simulink model "ieee14_fault"  (R2025b)
settings: Solver=ode23t  StartTime=0.0  StopTime=0.12  FixedStep=0.2  RelTol=1e-4  AbsTol=1e-6  EnableMultiTasking=on
undefined symbols (not defined in the file or in its folder): D1, Delta
libraries: spsDiodeLib x84, spsGroundLib x84, spsSeriesRLCBranchLib x84, spsDCVoltageSourceLib x84, spsBreakerLib x42, spsThreePhaseSeriesRLCBranchLib x20, spsThreePhaseVIMeasurementLib x16, spsThreePhaseFaultLib x14, spsThreePhaseSeriesRLCLoadLib x11, spsThreePhaseSourceLib x5, spsThreePhaseTransformerTwoWindingsLib x5, spspowerguiLib x1
(part 1 of 3)
settings Model: Creator=Bharath  LastModifiedBy=ubuntu
settings SolverCC: AutoScaleAbsTol=off  MaxConsecutiveMinStep=auto  ZeroCrossControl=DisableAll  AlgebraicLoopSolver=TrustRegion
settings DataIOCC: LimitDataPoints=on  SaveFormat=Array  SignalLoggingSaveFormat=ModelDataLogs  ReturnWorkspaceOutputs=off
settings OptimizationCC: ExpressionDepthLimit=2147483647.0  LifeSpan=inf
settings DebuggingCC: UnderspecifiedInitializationDetection=Classic  MergeDetectMultiDrivingBlocksExec=none  FcnCallInpInsideContextMsg=warning  UnconnectedInputMsg=warning  UnconnectedLineMsg=warning  StateNameClashWarn=warning  SFUnexpectedBacktrackingDiag=warning  SFNoUnconditionalDefaultTransitionDiag=warning  SFExecutionAtInitializationDiag=none  ArithmeticOperatorsInVariantConditions=warning
settings HardwareCC: ProdBitPerPointer=32.0  ProdBitPerSizeT=32.0  ProdBitPerPtrDiffT=32.0  ProdLargestAtomicFloat=None  ProdIntDivRoundTo=Undefined  ProdEndianess=Unspecified  ProdWordSize=32.0  ProdHWDeviceType=32-bit Generic
settings ModelReferenceCC: PropagateSignalLabelsOutOfModel=off
settings SFSimCC: SimUseLocalCustomCode=off  CustomCodeUndefinedFunction=UseInterfaceOnly
settings RTWCC: RTWUseLocalCustomCode=off  GPUComputeCapability=3.5
settings CodeAppCC: StateflowObjectComments=on
settings GRTTargetCC: TargetLangStandard=C89/C90 (ANSI)  CombineOutputUpdateFcns=off  GRTInterface=on
settings ConfigComp: CovMetricSettings=dw  CovSaveCumulativeToWorkspaceVar=on  CovSaveSingleToWorkspaceVar=on  CovExternalEMLEnable=off
settings SimscapeCC: SimscapeNormalizeSystem=off

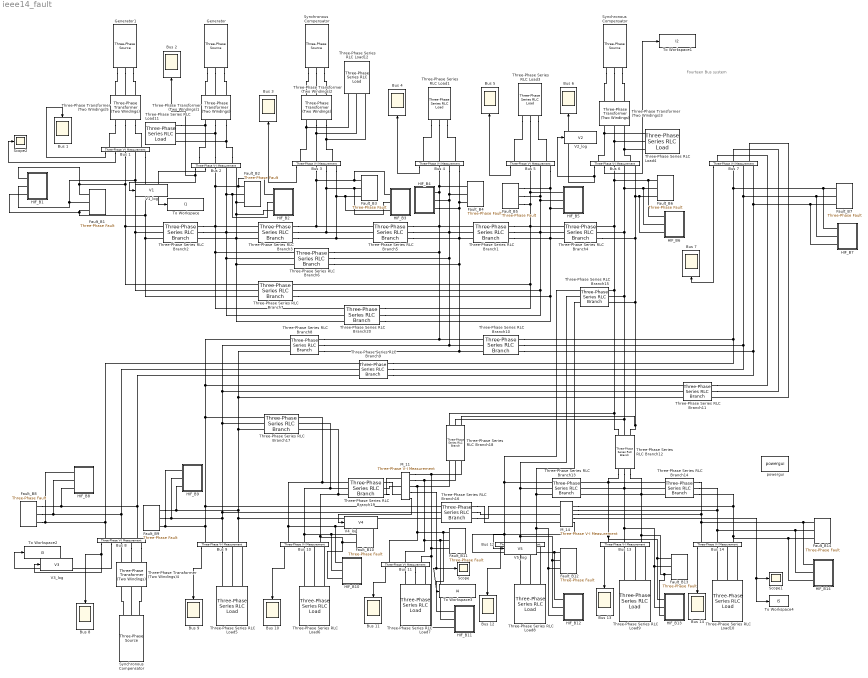
== system ieee14_fault ==
  note: Fourteen Bus system
  Bus {1..14} (14 alike) : Scope
      Bus 1 settings: TimeSpan=0.12  ActiveDisplayYMinimum=-239452.80918454356  ActiveDisplayYMaximum=239452.80923448486
      Bus 10 settings: TimeSpan=0.12  ActiveDisplayYMinimum=-309827.02088933904  ActiveDisplayYMaximum=309827.02017740381  DataLoggingVariableName=ScopeData9
      Bus 11 settings: TimeSpan=0.12  ActiveDisplayYMinimum=-231376.67698890329  ActiveDisplayYMaximum=231376.67636895  DataLoggingVariableName=ScopeData10
      Bus 12 settings: TimeSpan=0.12  ActiveDisplayYMinimum=-232519.39919438146  ActiveDisplayYMaximum=232519.39950023073  DataLoggingVariableName=ScopeData11
      Bus 13 settings: TimeSpan=0.12  ActiveDisplayYMinimum=-230979.08628975169  ActiveDisplayYMaximum=230979.08708078947  DataLoggingVariableName=ScopeData12
      Bus 14 settings: TimeSpan=0.12  ActiveDisplayYMinimum=-225636.53954069025  ActiveDisplayYMaximum=225636.53866563851  DataLoggingVariableName=ScopeData13
      Bus 2 settings: TimeSpan=0.12  ActiveDisplayYMinimum=171914.54239626692  ActiveDisplayYMaximum=195035.37027362009
      Bus 3 settings: TimeSpan=0.12  ActiveDisplayYMinimum=-230702.92082942094  ActiveDisplayYMaximum=230702.92067850774  DataLoggingVariableName=ScopeData6
      Bus 4 settings: TimeSpan=0.12  ActiveDisplayYMinimum=-233675.94578463773  ActiveDisplayYMaximum=233675.94517916857  DataLoggingVariableName=ScopeData2
      Bus 5 settings: TimeSpan=0.12  ActiveDisplayYMinimum=-234990.24443535894  ActiveDisplayYMaximum=234990.24383449319  DataLoggingVariableName=ScopeData3
      Bus 6 settings: TimeSpan=0.12  ActiveDisplayYMinimum=-236352.07231998953  ActiveDisplayYMaximum=236352.07224703734  DataLoggingVariableName=ScopeData5
      Bus 7 settings: TimeSpan=0.12  ActiveDisplayYMinimum=-301809.56696559861  ActiveDisplayYMaximum=301809.56695235  DataLoggingVariableName=ScopeData4
      Bus 8 settings: TimeSpan=0.12  ActiveDisplayYMinimum=-243227.45890859389  ActiveDisplayYMaximum=243227.4593976411  DataLoggingVariableName=ScopeData7
      Bus 9 settings: TimeSpan=0.12  ActiveDisplayYMinimum=-229028.21128421329  ActiveDisplayYMaximum=229028.21145489725  DataLoggingVariableName=ScopeData8
  "Bus 1 " : spsThreePhaseVIMeasurementLib/Three-Phase V-I Measurement  VoltageMeasurement=phase-to-ground  SetLabelV=off  LabelV=Vabc  Vpu=off  VpuLL=off  CurrentMeasurement=yes  SetLabelI=off  LabelI=Iabc  Ipu=off  Pbase=100e6  Vbase=0.95  OutputType=Complex  PhasorSimulation=off  PSBequivalent=0
  "Bus 10 " : spsThreePhaseVIMeasurementLib/Three-Phase V-I Measurement  VoltageMeasurement=phase-to-ground  SetLabelV=off  LabelV=Vabc  Vpu=off  VpuLL=off  CurrentMeasurement=yes  SetLabelI=off  LabelI=Iabc  Ipu=off  Pbase=100e6  Vbase=0.94  OutputType=Complex  PhasorSimulation=off  PSBequivalent=0
  "Bus 11 " : spsThreePhaseVIMeasurementLib/Three-Phase V-I Measurement  VoltageMeasurement=phase-to-ground  SetLabelV=off  LabelV=Vabc  Vpu=off  VpuLL=off  CurrentMeasurement=yes  SetLabelI=off  LabelI=Iabc  Ipu=off  Pbase=100e6  Vbase=0.95  OutputType=Complex  PhasorSimulation=off  PSBequivalent=0
  "Bus 12 " : spsThreePhaseVIMeasurementLib/Three-Phase V-I Measurement  VoltageMeasurement=phase-to-ground  SetLabelV=off  LabelV=Vabc  Vpu=off  VpuLL=off  CurrentMeasurement=yes  SetLabelI=off  LabelI=Iabc  Ipu=off  Pbase=100e6  Vbase=0.95  OutputType=Complex  PhasorSimulation=off  PSBequivalent=0
  "Bus 13 " : spsThreePhaseVIMeasurementLib/Three-Phase V-I Measurement  VoltageMeasurement=phase-to-ground  SetLabelV=off  LabelV=Vabc  Vpu=off  VpuLL=off  CurrentMeasurement=yes  SetLabelI=off  LabelI=Iabc  Ipu=off  Pbase=100e6  Vbase=0.95  OutputType=Complex  PhasorSimulation=off  PSBequivalent=0
  "Bus 14 " : spsThreePhaseVIMeasurementLib/Three-Phase V-I Measurement  VoltageMeasurement=phase-to-ground  SetLabelV=off  LabelV=Vabc  Vpu=off  VpuLL=off  CurrentMeasurement=yes  SetLabelI=off  LabelI=Iabc  Ipu=off  Pbase=100e6  Vbase=0.92  OutputType=Complex  PhasorSimulation=off  PSBequivalent=0
  "Bus 2 " : spsThreePhaseVIMeasurementLib/Three-Phase V-I Measurement  VoltageMeasurement=phase-to-ground  SetLabelV=off  LabelV=Vabc  Vpu=off  VpuLL=off  CurrentMeasurement=yes  SetLabelI=off  LabelI=Iabc  Ipu=off  Pbase=100e6  Vbase=0.95  OutputType=Complex  PhasorSimulation=off  PSBequivalent=0
  "Bus 3 " : spsThreePhaseVIMeasurementLib/Three-Phase V-I Measurement  VoltageMeasurement=phase-to-ground  SetLabelV=off  LabelV=Vabc  Vpu=off  VpuLL=off  CurrentMeasurement=yes  SetLabelI=off  LabelI=Iabc  Ipu=off  Pbase=100e6  Vbase=0.95  OutputType=Complex  PhasorSimulation=off  PSBequivalent=0
  "Bus 4 " : spsThreePhaseVIMeasurementLib/Three-Phase V-I Measurement  VoltageMeasurement=phase-to-ground  SetLabelV=off  LabelV=Vabc  Vpu=off  VpuLL=off  CurrentMeasurement=yes  SetLabelI=off  LabelI=Iabc  Ipu=off  Pbase=100e6  Vbase=0.95  OutputType=Complex  PhasorSimulation=off  PSBequivalent=0
  "Bus 5 " : spsThreePhaseVIMeasurementLib/Three-Phase V-I Measurement  VoltageMeasurement=phase-to-ground  SetLabelV=off  LabelV=Vabc  Vpu=off  VpuLL=off  CurrentMeasurement=yes  SetLabelI=off  LabelI=Iabc  Ipu=off  Pbase=100e6  Vbase=0.95  OutputType=Complex  PhasorSimulation=off  PSBequivalent=0
  "Bus 6 " : spsThreePhaseVIMeasurementLib/Three-Phase V-I Measurement  VoltageMeasurement=phase-to-ground  SetLabelV=off  LabelV=Vabc  Vpu=off  VpuLL=off  CurrentMeasurement=yes  SetLabelI=off  LabelI=Iabc  Ipu=off  Pbase=100e6  Vbase=0.95  OutputType=Complex  PhasorSimulation=off  PSBequivalent=0
  "Bus 7 " : spsThreePhaseVIMeasurementLib/Three-Phase V-I Measurement  VoltageMeasurement=phase-to-ground  SetLabelV=off  LabelV=Vabc  Vpu=off  VpuLL=off  CurrentMeasurement=yes  SetLabelI=off  LabelI=Iabc  Ipu=off  Pbase=100e6  Vbase=0.95  OutputType=Complex  PhasorSimulation=off  PSBequivalent=0
  "Bus 8 " : spsThreePhaseVIMeasurementLib/Three-Phase V-I Measurement  VoltageMeasurement=phase-to-ground  SetLabelV=off  LabelV=Vabc  Vpu=off  VpuLL=off  CurrentMeasurement=yes  SetLabelI=off  LabelI=Iabc  Ipu=off  Pbase=100e6  Vbase=1  OutputType=Complex  PhasorSimulation=off  PSBequivalent=0
  "Bus 9 " : spsThreePhaseVIMeasurementLib/Three-Phase V-I Measurement  VoltageMeasurement=phase-to-ground  SetLabelV=off  LabelV=Vabc  Vpu=off  VpuLL=off  CurrentMeasurement=yes  SetLabelI=off  LabelI=Iabc  Ipu=off  Pbase=100e6  Vbase=0.94  OutputType=Complex  PhasorSimulation=off  PSBequivalent=0
  Fault_B{1..14} (14 alike) : spsThreePhaseFaultLib/Three-Phase Fault  InitialStates=0  FaultA=on  FaultB=on  FaultC=on  GroundFault=on  SwitchTimes=[100]  External=off  SwitchStatus=NaN  FaultResistance=40  GroundResistance=40  SnubberResistance=1e6  SnubberCapacitance=inf  Measurements=None
  Generator : spsThreePhaseSourceLib/Three-Phase Source  InternalConnection=Yg  VoltagePhases=off  Voltage=240.35e3  PhaseAngle=-30  Voltage_phases=[25e3 25e3 25e3]/sqrt(3)  PhaseAngles_phases=[0 -120 +120]  Frequency=60  NonIdealSource=on  SpecifyImpedance=on  Resistance=0.8929  Inductance=16.58e-3  ShortCircuitLevel=2000e6  BaseVoltage=230e3  XRratio=10  BusType=PV  Pref=0.4  Qref=0  Prefabc=[10e3, 10e3, 10e3]  Qrefabc=[0, 0, 0]  Qmin=-0.4  Qmax=0.5
  Generator1 : spsThreePhaseSourceLib/Three-Phase Source  InternalConnection=Yg  VoltagePhases=off  Voltage=243.8e3  PhaseAngle=-30  Voltage_phases=[25e3 25e3 25e3]/sqrt(3)  PhaseAngles_phases=[0 -120 +120]  Frequency=60  NonIdealSource=on  SpecifyImpedance=on  Resistance=0.8929  Inductance=16.58e-3  ShortCircuitLevel=2000e6  BaseVoltage=230e3  XRratio=10  BusType=PQ  Pref=2.324  Qref=-0.169  Prefabc=[10e3, 10e3, 10e3]  Qrefabc=[0, 0, 0]  Qmin=0  Qmax=0
  HIF_B1 : Subsystem
  HIF_B10 : Subsystem
  HIF_B11 : Subsystem
  HIF_B12 : Subsystem
  HIF_B13 : Subsystem
  HIF_B14 : Subsystem
  HIF_B2 : Subsystem
  HIF_B3 : Subsystem
  HIF_B4 : Subsystem
  HIF_B5 : Subsystem
  HIF_B6 : Subsystem
  HIF_B7 : Subsystem
  HIF_B8 : Subsystem
  HIF_B9 : Subsystem
  M_11 : spsThreePhaseVIMeasurementLib/Three-Phase V-I Measurement  VoltageMeasurement=phase-to-ground  SetLabelV=off  LabelV=Vabc  Vpu=off  VpuLL=off  CurrentMeasurement=yes  SetLabelI=off  LabelI=Iabc  Ipu=off  Pbase=100e6  Vbase=0.95  OutputType=Complex  PhasorSimulation=off  PSBequivalent=0
  M_14 : spsThreePhaseVIMeasurementLib/Three-Phase V-I Measurement  VoltageMeasurement=phase-to-ground  SetLabelV=off  LabelV=Vabc  Vpu=off  VpuLL=off  CurrentMeasurement=yes  SetLabelI=off  LabelI=Iabc  Ipu=off  Pbase=100e6  Vbase=0.92  OutputType=Complex  PhasorSimulation=off  PSBequivalent=0
  Scope : Scope
      settings: ActiveDisplayYMinimum=-1  ActiveDisplayYMaximum=1  DataLoggingVariableName=ScopeData14
  Scope1 : Scope
      settings: ActiveDisplayYMinimum=-1  ActiveDisplayYMaximum=1  DataLoggingVariableName=ScopeData15
  Scope2 : Scope
      settings: ActiveDisplayYMinimum=-1  ActiveDisplayYMaximum=1  DataLoggingVariableName=ScopeData16
  Synchronous  Compensator : spsThreePhaseSourceLib/Three-Phase Source  InternalConnection=Yg  VoltagePhases=off  Voltage=232.3e3  PhaseAngle=-30  Voltage_phases=[25e3 25e3 25e3]/sqrt(3)  PhaseAngles_phases=[0 -120 +120]  Frequency=60  NonIdealSource=on  SpecifyImpedance=on  Resistance=0.8929  Inductance=16.58e-3  ShortCircuitLevel=2000e6  BaseVoltage=230e3  XRratio=10  BusType=PV  Pref=0  Qref=23.4e6  Prefabc=[10e3, 10e3, 10e3]  Qrefabc=[0, 0, 0]  Qmin=0  Qmax=0.4
  "Synchronous  Compensator " : spsThreePhaseSourceLib/Three-Phase Source  InternalConnection=Yg  VoltagePhases=off  Voltage=246.1e3  PhaseAngle=-30  Voltage_phases=[25e3 25e3 25e3]/sqrt(3)  PhaseAngles_phases=[0 -120 +120]  Frequency=60  NonIdealSource=on  SpecifyImpedance=on  Resistance=0.8929  Inductance=16.58e-3  ShortCircuitLevel=2000e6  BaseVoltage=230e3  XRratio=10  BusType=PV  Pref=0  Qref=23.4e6  Prefabc=[10e3, 10e3, 10e3]  Qrefabc=[0, 0, 0]  Qmin=-0.06  Qmax=0.24
  Synchronous Compensator : spsThreePhaseSourceLib/Three-Phase Source  InternalConnection=Yg  VoltagePhases=off  Voltage=250.7e3  PhaseAngle=-30  Voltage_phases=[25e3 25e3 25e3]/sqrt(3)  PhaseAngles_phases=[0 -120 +120]  Frequency=60  NonIdealSource=on  SpecifyImpedance=on  Resistance=0.8929  Inductance=16.58e-3  ShortCircuitLevel=2000e6  BaseVoltage=230e3  XRratio=10  BusType=PV  Pref=0  Qref=0  Prefabc=[10e3, 10e3, 10e3]  Qrefabc=[0, 0, 0]  Qmin=-0.06  Qmax=0.24
  Three-Phase Series RLC Branch1 : spsThreePhaseSeriesRLCBranchLib/Three-Phase Series RLC Branch  LConnTagsString=A|B|C  RConnTagsString=A|B|C  BranchType=RL  Resistance=0.01335*529  Inductance=0.04211*529/(2*pi*60)  Capacitance=1/0.012*pi*60)  Measurements=None
  Three-Phase Series RLC Branch10 : spsThreePhaseSeriesRLCBranchLib/Three-Phase Series RLC Branch  LConnTagsString=A|B|C  RConnTagsString=A|B|C  BranchType=L  Resistance=1  Inductance=0.20912*529/(2*pi*60)  Capacitance=1e-6  Measurements=None
  Three-Phase Series RLC Branch11 : spsThreePhaseSeriesRLCBranchLib/Three-Phase Series RLC Branch  LConnTagsString=A|B|C  RConnTagsString=A|B|C  BranchType=L  Resistance=1  Inductance=0.11001*529/(2*pi*60)  Capacitance=1e-6  Measurements=None
  Three-Phase Series RLC Branch12 : spsThreePhaseSeriesRLCBranchLib/Three-Phase Series RLC Branch  LConnTagsString=A|B|C  RConnTagsString=A|B|C  BranchType=RL  Resistance=0.06615*529  Inductance=0.13027*529/(2*pi*60)  Capacitance=1e-6  Measurements=None
  Three-Phase Series RLC Branch13 : spsThreePhaseSeriesRLCBranchLib/Three-Phase Series RLC Branch  LConnTagsString=A|B|C  RConnTagsString=A|B|C  BranchType=RL  Resistance=0.22092*529  Inductance=0.19988*529/(2*pi*60)  Capacitance=1e-6  Measurements=None
  Three-Phase Series RLC Branch14 : spsThreePhaseSeriesRLCBranchLib/Three-Phase Series RLC Branch  LConnTagsString=A|B|C  RConnTagsString=A|B|C  BranchType=RL  Resistance=0.17093*529  Inductance=0.34802*529/(2*pi*60)  Capacitance=1e-6  Measurements=None
  Three-Phase Series RLC Branch15 : spsThreePhaseSeriesRLCBranchLib/Three-Phase Series RLC Branch  LConnTagsString=A|B|C  RConnTagsString=A|B|C  BranchType=RL  Resistance=0.12291*529  Inductance=0.25581*529/(2*pi*60)  Capacitance=1e-6  Measurements=None
  Three-Phase Series RLC Branch16 : spsThreePhaseSeriesRLCBranchLib/Three-Phase Series RLC Branch  LConnTagsString=A|B|C  RConnTagsString=A|B|C  BranchType=RL  Resistance=0.12711*529  Inductance=0.27038*529/(2*pi*60)  Capacitance=1e-6  Measurements=None
  Three-Phase Series RLC Branch17 : spsThreePhaseSeriesRLCBranchLib/Three-Phase Series RLC Branch  LConnTagsString=A|B|C  RConnTagsString=A|B|C  BranchType=RL  Resistance=0.03181*529  Inductance=0.08450*529/(2*pi*60)  Capacitance=1e-6  Measurements=None
  Three-Phase Series RLC Branch18 : spsThreePhaseSeriesRLCBranchLib/Three-Phase Series RLC Branch  LConnTagsString=A|B|C  RConnTagsString=A|B|C  BranchType=RL  Resistance=0.09498*529  Inductance=0.1989*529/(2*pi*60)  Capacitance=1e-6  Measurements=None
  Three-Phase Series RLC Branch19 : spsThreePhaseSeriesRLCBranchLib/Three-Phase Series RLC Branch  LConnTagsString=A|B|C  RConnTagsString=A|B|C  BranchType=RL  Resistance=0.08205*529  Inductance=0.19207*529/(2*pi*60)  Capacitance=1e-6  Measurements=None
  Three-Phase Series RLC Branch2 : spsThreePhaseSeriesRLCBranchLib/Three-Phase Series RLC Branch  LConnTagsString=A|B|C  RConnTagsString=A|B|C  BranchType=RL  Resistance=0.01938*529  Inductance=0.05917*529/(2*pi*60)  Capacitance=1/0.0528/(2*pi*50)  Measurements=None
  Three-Phase Series RLC Branch20 : spsThreePhaseSeriesRLCBranchLib/Three-Phase Series RLC Branch  LConnTagsString=A|B|C  RConnTagsString=A|B|C  BranchType=RL  Resistance=0.05695*529  Inductance=0.17388*529/(2*pi*60)  Capacitance=1/0.0340/(2*pi*50)  Measurements=None
  Three-Phase Series RLC Branch3 : spsThreePhaseSeriesRLCBranchLib/Three-Phase Series RLC Branch  LConnTagsString=A|B|C  RConnTagsString=A|B|C  BranchType=RL  Resistance=0.04699*529  Inductance=0.19797*529/(2*pi*60)  Capacitance=1/0.0438/(2*pi*50)  Measurements=None
  Three-Phase Series RLC Branch4 : spsThreePhaseSeriesRLCBranchLib/Three-Phase Series RLC Branch  LConnTagsString=A|B|C  RConnTagsString=A|B|C  BranchType=L  Resistance=1  Inductance=0.25202*529/(2*pi*60)  Capacitance=1e-6  Measurements=None
  Three-Phase Series RLC Branch5 : spsThreePhaseSeriesRLCBranchLib/Three-Phase Series RLC Branch  LConnTagsString=A|B|C  RConnTagsString=A|B|C  BranchType=RL  Resistance=0.06701*529  Inductance=0.17103*529/(2*pi*60)  Capacitance=1/0.0346/(2*pi*50)  Measurements=None
  Three-Phase Series RLC Branch6 : spsThreePhaseSeriesRLCBranchLib/Three-Phase Series RLC Branch  LConnTagsString=A|B|C  RConnTagsString=A|B|C  BranchType=RL  Resistance=0.05811*529  Inductance=0.17632*529/(2*pi*60)  Capacitance=1/0.0374/(2*pi*50)  Measurements=None
  Three-Phase Series RLC Branch7 : spsThreePhaseSeriesRLCBranchLib/Three-Phase Series RLC Branch  LConnTagsString=A|B|C  RConnTagsString=A|B|C  BranchType=RL  Resistance=0.05403*529  Inductance=0.22304*529/(2*pi*60)  Capacitance=1/0.0492/(2*pi*50)  Measurements=None
  Three-Phase Series RLC Branch8 : spsThreePhaseSeriesRLCBranchLib/Three-Phase Series RLC Branch  LConnTagsString=A|B|C  RConnTagsString=A|B|C  BranchType=L  Resistance=1  Inductance=0.55618*529/(2*pi*60)  Capacitance=1e-6  Measurements=None
  Three-Phase Series RLC Branch9 : spsThreePhaseSeriesRLCBranchLib/Three-Phase Series RLC Branch  LConnTagsString=A|B|C  RConnTagsString=A|B|C  BranchType=L  Resistance=1  Inductance=0.17615*529/(2*pi*60)  Capacitance=1e-6  Measurements=None
  Three-Phase Series RLC Load1 : spsThreePhaseSeriesRLCLoadLib/Three-Phase Series RLC Load  LConnTagsString=A|B|C  Configuration=Y (grounded)  NominalVoltage=230e3  Vabc=[1e3 1e3 1e3]  Vabcp=[1e3 1e3 1e3]  NominalFrequency=60  UnbalancedPower=off  ActivePower=47.8e6  InductivePower=0  CapacitivePower=3.9e6  Pabc=[10e3 9e3 11e3]  QLabc=[100 90 110]  QCabc=[100 90 110]  Pabcp=[10e3 9e3 11e3]  QLabcp=[100 90 110]  QCabcp=[100 90 110]  Measurements=None  LoadType=constant PQ
  Three-Phase Series RLC Load10 : spsThreePhaseSeriesRLCLoadLib/Three-Phase Series RLC Load  LConnTagsString=A|B|C  Configuration=Y (grounded)  NominalVoltage=230e3  Vabc=[1e3 1e3 1e3]  Vabcp=[1e3 1e3 1e3]  NominalFrequency=60  UnbalancedPower=off  ActivePower=14.9e6  InductivePower=5e6  CapacitivePower=0  Pabc=[10e3 9e3 11e3]  QLabc=[100 90 110]  QCabc=[100 90 110]  Pabcp=[10e3 9e3 11e3]  QLabcp=[100 90 110]  QCabcp=[100 90 110]  Measurements=None  LoadType=constant Z
  Three-Phase Series RLC Load11 : spsThreePhaseSeriesRLCLoadLib/Three-Phase Series RLC Load  LConnTagsString=A|B|C  Configuration=Y (grounded)  NominalVoltage=230e3  Vabc=[1e3 1e3 1e3]  Vabcp=[1e3 1e3 1e3]  NominalFrequency=60  UnbalancedPower=off  ActivePower=21.7e6  InductivePower=12.7e6  CapacitivePower=0  Pabc=[10e3 9e3 11e3]  QLabc=[100 90 110]  QCabc=[100 90 110]  Pabcp=[10e3 9e3 11e3]  QLabcp=[100 90 110]  QCabcp=[100 90 110]  Measurements=Branch currents  LoadType=constant PQ
  Three-Phase Series RLC Load12 : spsThreePhaseSeriesRLCLoadLib/Three-Phase Series RLC Load  LConnTagsString=A|B|C  Configuration=Y (grounded)  NominalVoltage=230e3  Vabc=[1e3 1e3 1e3]  Vabcp=[1e3 1e3 1e3]  NominalFrequency=60  UnbalancedPower=off  ActivePower=94.2e6  InductivePower=19e6  CapacitivePower=0  Pabc=[10e3 9e3 11e3]  QLabc=[100 90 110]  QCabc=[100 90 110]  Pabcp=[10e3 9e3 11e3]  QLabcp=[100 90 110]  QCabcp=[100 90 110]  Measurements=None  LoadType=constant PQ
  Three-Phase Series RLC Load3 : spsThreePhaseSeriesRLCLoadLib/Three-Phase Series RLC Load  LConnTagsString=A|B|C  Configuration=Y (grounded)  NominalVoltage=230e3  Vabc=[1e3 1e3 1e3]  Vabcp=[1e3 1e3 1e3]  NominalFrequency=60  UnbalancedPower=off  ActivePower=7.6e6  InductivePower=1.6e6  CapacitivePower=0  Pabc=[10e3 9e3 11e3]  QLabc=[100 90 110]  QCabc=[100 90 110]  Pabcp=[10e3 9e3 11e3]  QLabcp=[100 90 110]  QCabcp=[100 90 110]  Measurements=None  LoadType=constant PQ
  Three-Phase Series RLC Load4 : spsThreePhaseSeriesRLCLoadLib/Three-Phase Series RLC Load  LConnTagsString=A|B|C  Configuration=Y (grounded)  NominalVoltage=230e3  Vabc=[1e3 1e3 1e3]  Vabcp=[1e3 1e3 1e3]  NominalFrequency=60  UnbalancedPower=off  ActivePower=11.2e6  InductivePower=7.5e6  CapacitivePower=0  Pabc=[10e3 9e3 11e3]  QLabc=[100 90 110]  QCabc=[100 90 110]  Pabcp=[10e3 9e3 11e3]  QLabcp=[100 90 110]  QCabcp=[100 90 110]  Measurements=None  LoadType=constant PQ
  Three-Phase Series RLC Load5 : spsThreePhaseSeriesRLCLoadLib/Three-Phase Series RLC Load  LConnTagsString=A|B|C  Configuration=Y (grounded)  NominalVoltage=230e3  Vabc=[1e3 1e3 1e3]  Vabcp=[1e3 1e3 1e3]  NominalFrequency=60  UnbalancedPower=off  ActivePower=29.5e6  InductivePower=16.6e6  CapacitivePower=0  Pabc=[10e3 9e3 11e3]  QLabc=[100 90 110]  QCabc=[100 90 110]  Pabcp=[10e3 9e3 11e3]  QLabcp=[100 90 110]  QCabcp=[100 90 110]  Measurements=None  LoadType=constant PQ
  Three-Phase Series RLC Load6 : spsThreePhaseSeriesRLCLoadLib/Three-Phase Series RLC Load  LConnTagsString=A|B|C  Configuration=Y (grounded)  NominalVoltage=230e3  Vabc=[1e3 1e3 1e3]  Vabcp=[1e3 1e3 1e3]  NominalFrequency=60  UnbalancedPower=off  ActivePower=9e6  InductivePower=5.8e6  CapacitivePower=0  Pabc=[10e3 9e3 11e3]  QLabc=[100 90 110]  QCabc=[100 90 110]  Pabcp=[10e3 9e3 11e3]  QLabcp=[100 90 110]  QCabcp=[100 90 110]  Measurements=None  LoadType=constant PQ
  Three-Phase Series RLC Load7 : spsThreePhaseSeriesRLCLoadLib/Three-Phase Series RLC Load  LConnTagsString=A|B|C  Configuration=Y (grounded)  NominalVoltage=230e3  Vabc=[1e3 1e3 1e3]  Vabcp=[1e3 1e3 1e3]  NominalFrequency=60  UnbalancedPower=off  ActivePower=3.5e6  InductivePower=1.8e6  CapacitivePower=0  Pabc=[10e3 9e3 11e3]  QLabc=[100 90 110]  QCabc=[100 90 110]  Pabcp=[10e3 9e3 11e3]  QLabcp=[100 90 110]  QCabcp=[100 90 110]  Measurements=None  LoadType=constant PQ
  Three-Phase Series RLC Load8 : spsThreePhaseSeriesRLCLoadLib/Three-Phase Series RLC Load  LConnTagsString=A|B|C  Configuration=Y (grounded)  NominalVoltage=230e3  Vabc=[1e3 1e3 1e3]  Vabcp=[1e3 1e3 1e3]  NominalFrequency=60  UnbalancedPower=off  ActivePower=6.1e6  InductivePower=1.6e6  CapacitivePower=0  Pabc=[10e3 9e3 11e3]  QLabc=[100 90 110]  QCabc=[100 90 110]  Pabcp=[10e3 9e3 11e3]  QLabcp=[100 90 110]  QCabcp=[100 90 110]  Measurements=None  LoadType=constant PQ
  Three-Phase Series RLC Load9 : spsThreePhaseSeriesRLCLoadLib/Three-Phase Series RLC Load  LConnTagsString=A|B|C  Configuration=Y (grounded)  NominalVoltage=230e3  Vabc=[1e3 1e3 1e3]  Vabcp=[1e3 1e3 1e3]  NominalFrequency=60  UnbalancedPower=off  ActivePower=13.5e6  InductivePower=5.8e6  CapacitivePower=0  Pabc=[10e3 9e3 11e3]  QLabc=[100 90 110]  QCabc=[100 90 110]  Pabcp=[10e3 9e3 11e3]  QLabcp=[100 90 110]  QCabcp=[100 90 110]  Measurements=None  LoadType=constant PQ
  Three-Phase Transformer (Two Windings)1 : spsThreePhaseTransformerTwoWindingsLib/Three-Phase Transformer (Two Windings)  Winding1Connection=Delta (D1)  Winding2Connection=Yg  CoreType=Three single-phase transformers  SetSaturation=off  Hysteresis=off  DataFile='hysteresis'  SetInitialFlux=off  Measurements=None  UNITS=pu  NominalPower=[ 100e6 , 60 ]  Winding1=[ 230e3 , 0.002 , 0.08 ]  Winding2=[ 230e3 , 0.002 , 0.08 ]  Rm=500  Lm=500  L0=0.5  Saturation=[ 0,0 ; 0.0024,1.2 ; 1.0,1.52 ]  InitialFluxes=[ 0.8 , -0.8 , 0.7 ]  BreakLoop=off  DiscreteSolver=Trapezoidal iterative  DataType=off  TransfoNumber=1
  Three-Phase Transformer (Two Windings)2 : spsThreePhaseTransformerTwoWindingsLib/Three-Phase Transformer (Two Windings)  Winding1Connection=Delta (D1)  Winding2Connection=Yg  CoreType=Three single-phase transformers  SetSaturation=off  Hysteresis=off  DataFile='hysteresis'  SetInitialFlux=off  Measurements=None  UNITS=pu  NominalPower=[ 100e6 , 60 ]  Winding1=[ 230e3 , 0.002 , 0.08 ]  Winding2=[ 230e3 , 0.002 , 0.08 ]  Rm=500  Lm=500  L0=0.5  Saturation=[ 0,0 ; 0.0024,1.2 ; 1.0,1.52 ]  InitialFluxes=[ 0.8 , -0.8 , 0.7 ]  BreakLoop=off  DiscreteSolver=Trapezoidal iterative  DataType=off  TransfoNumber=1
  Three-Phase Transformer (Two Windings)3 : spsThreePhaseTransformerTwoWindingsLib/Three-Phase Transformer (Two Windings)  Winding1Connection=Delta (D1)  Winding2Connection=Yg  CoreType=Three single-phase transformers  SetSaturation=off  Hysteresis=off  DataFile='hysteresis'  SetInitialFlux=off  Measurements=None  UNITS=pu  NominalPower=[ 100e6 , 60 ]  Winding1=[ 230e3 , 0.002 , 0.08 ]  Winding2=[ 230e3 , 0.002 , 0.08 ]  Rm=500  Lm=500  L0=0.5  Saturation=[ 0,0 ; 0.0024,1.2 ; 1.0,1.52 ]  InitialFluxes=[ 0.8 , -0.8 , 0.7 ]  BreakLoop=off  DiscreteSolver=Trapezoidal iterative  DataType=off  TransfoNumber=1
  Three-Phase Transformer (Two Windings)4 : spsThreePhaseTransformerTwoWindingsLib/Three-Phase Transformer (Two Windings)  Winding1Connection=Yg  Winding2Connection=Delta (D1)  CoreType=Three single-phase transformers  SetSaturation=off  Hysteresis=off  DataFile='hysteresis'  SetInitialFlux=off  Measurements=None  UNITS=pu  NominalPower=[ 100e6 , 60 ]  Winding1=[ 230e3 , 0.002 , 0.08 ]  Winding2=[ 230e3 , 0.002 , 0.08 ]  Rm=500  Lm=500  L0=0.5  Saturation=[0 0;0.0023999 1.2;1 1.52]  InitialFluxes=[0.80002 -0.80002 0.69999]  BreakLoop=off  DiscreteSolver=Trapezoidal iterative  DataType=off  TransfoNumber=1
  Three-Phase Transformer (Two Windings)5 : spsThreePhaseTransformerTwoWindingsLib/Three-Phase Transformer (Two Windings)  Winding1Connection=Delta (D1)  Winding2Connection=Yg  CoreType=Three single-phase transformers  SetSaturation=off  Hysteresis=off  DataFile='hysteresis'  SetInitialFlux=off  Measurements=None  UNITS=pu  NominalPower=[ 100e6 , 60 ]  Winding1=[ 230e3, 0.002, 0.08 ]  Winding2=[ 230e3 , 0.002 , 0.08 ]  Rm=500  Lm=500  L0=0.5  Saturation=[ 0,0 ; 0.0024,1.2 ; 1.0,1.52 ]  InitialFluxes=[ 0.8 , -0.8 , 0.7 ]  BreakLoop=off  DiscreteSolver=Trapezoidal iterative  DataType=off  TransfoNumber=1
  To Workspace : ToWorkspace  VariableName=I1  SaveFormat=Structure With Time  SampleTime=-1
  To Workspace1 : ToWorkspace  VariableName=I2  SaveFormat=Structure With Time  SampleTime=-1
  To Workspace2 : ToWorkspace  VariableName=I3  SaveFormat=Structure With Time  SampleTime=-1
  To Workspace3 : ToWorkspace  VariableName=I4  SaveFormat=Structure With Time  SampleTime=-1
  To Workspace4 : ToWorkspace  VariableName=I5  SaveFormat=Structure With Time  SampleTime=-1
  V1_log : ToWorkspace  VariableName=V1  SaveFormat=Structure With Time  SampleTime=1.3e-6
  V2_log : ToWorkspace  VariableName=V2  SaveFormat=Structure With Time  SampleTime=1.3e-6
  V3_log : ToWorkspace  VariableName=V3  SaveFormat=Structure With Time  SampleTime=1.3e-6
  V4_log : ToWorkspace  VariableName=V4  SaveFormat=Structure With Time  SampleTime=1.3e-6
  V5_log : ToWorkspace  VariableName=V5  SaveFormat=Structure With Time  SampleTime=1.3e-6
  powergui : spspowerguiLib/powergui  Priority=1  SimulationMode=Discrete  SampleTime=1.3e-6  frequency=60  Iterations=50  frequencyindice=60  Pbase=100e6  ErrMax=1e-4  UnitsV=kV  UnitsW=MW  buscounter=0  FunctionMessages=off  echomessages=off  EnableUseOfTLC=off  CurrentSourceSwitches=on  DisableSnubberDevices=off  DisableRonSwitches=off  DisableVfSwitches=off  DisplayEquations=off  AutomaticDiscreteSolvers=off  SolverType=Tustin  Interpol=off  ExternalGateDelay=off  methode=off  Ts=100  x0status=blocks  SPID=off  SwTol=0  HookPort=off  NonlinearTolerance=1e-4  nMaxIteration=100  ContinueOnMaxIteration=off  RestoreLinks=warning  ResistiveCurrentMeasurement=off  Frange=[0:2:500]  Ylog=off  Xlog=on  ShowGrid=off  save=off  variable=ZData  structure=0  ZoomFFT=off  StartTime=0.0  cycles=1  DisplayStyle=1  fundamental=60  FreqAxis=off  MaxFrequency=1000  frequencyindicesteady=1  RmsSteady=1  display=off
  wires:
  "Bus 11 "/1 -> Bus 11/1
  "Bus 10 "/1 -> Bus 10/1
  "Bus 9 "/1 -> Bus 9/1
  "Bus 8 "/1 -> Bus 8/1, V3_log/1
  "Bus 7 "/1 -> Bus 7/1
  "Bus 4 "/1 -> Bus 4/1
  "Bus 2 "/1 -> Bus 2/1, V1_log/1
  "Bus 14 "/1 -> Bus 14/1
  "Bus 13 "/1 -> Bus 13/1
  "Bus 12 "/1 -> Bus 12/1
  "Bus 5 "/1 -> Bus 5/1
  "Bus 1 "/1 -> Bus 1/1
  "Bus 3 "/1 -> Bus 3/1
  "Bus 6 "/1 -> Bus 6/1, V2_log/1
  "Bus 2 "/2 -> To Workspace/1
  "Bus 6 "/2 -> To Workspace1/1
  "Bus 8 "/2 -> To Workspace2/1
  M_11/2 -> Scope/1, To Workspace3/1
  M_14/2 -> To Workspace4/1, Scope1/1
  "Bus 1 "/2 -> Scope2/1
  M_11/1 -> V4_log/1
  M_14/1 -> V5_log/1
  connections:
  Three-Phase Series RLC Branch16/RConn3 -- HIF_B9/LConn3 -- Fault_B9/LConn3 -- Three-Phase Series RLC Branch17/RConn3 -- Three-Phase Series RLC Branch11/RConn3 -- Three-Phase Series RLC Branch8/LConn3 -- "Bus 9 "/LConn3
  HIF_B9/LConn2 -- Fault_B9/LConn2 -- "Bus 9 "/LConn2 -- Three-Phase Series RLC Branch16/RConn2 -- Three-Phase Series RLC Branch17/RConn2 -- Three-Phase Series RLC Branch11/RConn2 -- Three-Phase Series RLC Branch8/LConn2
  Three-Phase Series RLC Branch16/RConn1 -- HIF_B9/LConn1 -- Fault_B9/LConn1 -- "Bus 9 "/LConn1 -- Three-Phase Series RLC Branch17/RConn1 -- Three-Phase Series RLC Branch11/RConn1 -- Three-Phase Series RLC Branch8/LConn1
  Three-Phase Series RLC Branch10/RConn3 -- Three-Phase Series RLC Branch9/RConn3 -- HIF_B7/LConn3 -- Fault_B7/LConn3 -- "Bus 7 "/RConn3
  Three-Phase Series RLC Branch10/RConn2 -- Three-Phase Series RLC Branch9/RConn2 -- HIF_B7/LConn2 -- Fault_B7/LConn2 -- "Bus 7 "/RConn2
  Three-Phase Series RLC Branch10/RConn1 -- Three-Phase Series RLC Branch9/RConn1 -- HIF_B7/LConn1 -- Fault_B7/LConn1 -- "Bus 7 "/RConn1
  Three-Phase Series RLC Branch4/RConn3 -- Three-Phase Series RLC Branch12/LConn3 -- Three-Phase Series RLC Branch18/LConn3 -- Three-Phase Series RLC Branch15/LConn3 -- HIF_B6/LConn3 -- Fault_B6/LConn3 -- "Bus 6 "/RConn3
  Three-Phase Series RLC Branch15/LConn2 -- Three-Phase Series RLC Branch18/LConn2 -- Three-Phase Series RLC Branch12/LConn2 -- Three-Phase Series RLC Branch4/RConn2 -- HIF_B6/LConn2 -- Fault_B6/LConn2 -- "Bus 6 "/RConn2
  Three-Phase Series RLC Branch12/LConn1 -- Three-Phase Series RLC Branch18/LConn1 -- Three-Phase Series RLC Branch15/LConn1 -- Three-Phase Series RLC Branch4/RConn1 -- HIF_B6/LConn1 -- Fault_B6/LConn1 -- "Bus 6 "/RConn1
  "Bus 5 "/RConn3 -- Fault_B5/LConn3 -- HIF_B5/LConn3 -- Three-Phase Series RLC Branch1/RConn3 -- Three-Phase Series RLC Branch20/RConn3 -- Three-Phase Series RLC Branch7/RConn3 -- Three-Phase Series RLC Branch4/LConn3
  Three-Phase Series RLC Branch1/RConn2 -- Three-Phase Series RLC Branch20/RConn2 -- Three-Phase Series RLC Branch7/RConn2 -- Three-Phase Series RLC Branch4/LConn2 -- HIF_B5/LConn2 -- "Bus 5 "/RConn2 -- Fault_B5/LConn2
  Three-Phase Series RLC Branch1/RConn1 -- Three-Phase Series RLC Branch20/RConn1 -- Three-Phase Series RLC Branch7/RConn1 -- Three-Phase Series RLC Branch4/LConn1 -- Fault_B5/LConn1 -- HIF_B5/LConn1 -- "Bus 5 "/RConn1
  "Bus 3 "/RConn2 -- HIF_B3/LConn2 -- Fault_B3/LConn2 -- Three-Phase Series RLC Branch5/LConn2 -- Three-Phase Series RLC Branch3/RConn2
  "Bus 3 "/RConn1 -- HIF_B3/LConn1 -- Fault_B3/LConn1 -- Three-Phase Series RLC Branch5/LConn1 -- Three-Phase Series RLC Branch3/RConn1
  Three-Phase Series RLC Branch20/LConn3 -- Three-Phase Series RLC Branch6/LConn3 -- Three-Phase Series RLC Branch3/LConn3 -- Three-Phase Series RLC Branch2/RConn3 -- Fault_B2/LConn3 -- "Bus 2 "/RConn3 -- HIF_B2/LConn3
  Three-Phase Series RLC Branch20/LConn2 -- Three-Phase Series RLC Branch6/LConn2 -- Three-Phase Series RLC Branch2/RConn2 -- Three-Phase Series RLC Branch3/LConn2 -- HIF_B2/LConn2 -- Fault_B2/LConn2 -- "Bus 2 "/RConn2
  Three-Phase Series RLC Branch20/LConn1 -- Three-Phase Series RLC Branch6/LConn1 -- Three-Phase Series RLC Branch2/RConn1 -- Three-Phase Series RLC Branch3/LConn1 -- HIF_B2/LConn1 -- Fault_B2/LConn1 -- "Bus 2 "/RConn1
  "Bus 2 "/LConn2 -- Three-Phase Series RLC Load11/LConn2 -- Three-Phase Transformer (Two Windings)1/RConn2
  "Bus 2 "/LConn1 -- Three-Phase Series RLC Load11/LConn1 -- Three-Phase Transformer (Two Windings)1/RConn1
  Three-Phase Series RLC Branch14/LConn3 -- M_14/RConn3 -- HIF_B14/LConn3 -- Fault_B14/LConn3 -- "Bus 14 "/LConn3
  Three-Phase Series RLC Branch14/LConn2 -- M_14/RConn2 -- HIF_B14/LConn2 -- Fault_B14/LConn2 -- "Bus 14 "/LConn2
  Three-Phase Series RLC Branch14/LConn1 -- HIF_B14/LConn1 -- Fault_B14/LConn1 -- "Bus 14 "/LConn1 -- M_14/RConn1
  Three-Phase Series RLC Branch14/RConn3 -- Three-Phase Series RLC Branch13/LConn3 -- Three-Phase Series RLC Branch12/RConn3 -- HIF_B13/LConn3 -- Fault_B13/LConn3 -- "Bus 13 "/LConn3
  Three-Phase Series RLC Branch14/RConn2 -- Three-Phase Series RLC Branch12/RConn2 -- Three-Phase Series RLC Branch13/LConn2 -- HIF_B13/LConn2 -- Fault_B13/LConn2 -- "Bus 13 "/LConn2
  Three-Phase Series RLC Branch14/RConn1 -- Three-Phase Series RLC Branch12/RConn1 -- Three-Phase Series RLC Branch13/LConn1 -- HIF_B13/LConn1 -- Fault_B13/LConn1 -- "Bus 13 "/LConn1
  Three-Phase Series RLC Branch13/RConn3 -- Three-Phase Series RLC Branch15/RConn3 -- HIF_B12/LConn3 -- Fault_B12/LConn3 -- "Bus 12 "/LConn3
  Three-Phase Series RLC Branch13/RConn2 -- Three-Phase Series RLC Branch15/RConn2 -- HIF_B12/LConn2 -- Fault_B12/LConn2 -- "Bus 12 "/LConn2
  Three-Phase Series RLC Branch13/RConn1 -- Three-Phase Series RLC Branch15/RConn1 -- HIF_B12/LConn1 -- Fault_B12/LConn1 -- "Bus 12 "/LConn1
  Three-Phase Series RLC Branch17/LConn3 -- Three-Phase Series RLC Branch19/LConn3 -- HIF_B10/LConn3 -- Fault_B10/LConn3 -- "Bus 10 "/LConn3
  Three-Phase Series RLC Branch17/LConn2 -- Three-Phase Series RLC Branch19/LConn2 -- HIF_B10/LConn2 -- Fault_B10/LConn2 -- "Bus 10 "/LConn2
  Three-Phase Series RLC Branch17/LConn1 -- Three-Phase Series RLC Branch19/LConn1 -- HIF_B10/LConn1 -- Fault_B10/LConn1 -- "Bus 10 "/LConn1
  HIF_B1/LConn3 -- Fault_B1/LConn3 -- "Bus 1 "/RConn3 -- Three-Phase Series RLC Branch7/LConn3 -- Three-Phase Series RLC Branch2/LConn3
  HIF_B1/LConn2 -- Fault_B1/LConn2 -- "Bus 1 "/RConn2 -- Three-Phase Series RLC Branch7/LConn2 -- Three-Phase Series RLC Branch2/LConn2
  "Bus 1 "/RConn1 -- Fault_B1/LConn1 -- HIF_B1/LConn1 -- Three-Phase Series RLC Branch2/LConn1 -- Three-Phase Series RLC Branch7/LConn1
  Three-Phase Series RLC Load1/LConn3 -- "Bus 4 "/LConn3
  "Bus 8 "/RConn3 -- Three-Phase Transformer (Two Windings)4/LConn3
  "Bus 8 "/RConn2 -- Three-Phase Transformer (Two Windings)4/LConn2
  Three-Phase Transformer (Two Windings)4/LConn1 -- "Bus 8 "/RConn1
  Three-Phase Series RLC Load5/LConn2 -- "Bus 9 "/RConn2
  "Bus 9 "/RConn1 -- Three-Phase Series RLC Load5/LConn1
  Three-Phase Series RLC Load5/LConn3 -- "Bus 9 "/RConn3
  Generator/RConn2 -- Three-Phase Transformer (Two Windings)1/LConn2
  Three-Phase Series RLC Load1/LConn2 -- "Bus 4 "/LConn2
  Three-Phase Series RLC Load3/LConn1 -- "Bus 5 "/LConn1
  Three-Phase Series RLC Load3/LConn3 -- "Bus 5 "/LConn3
  "Bus 7 "/LConn3 -- Three-Phase Series RLC Branch11/LConn3
  Three-Phase Series RLC Load3/LConn2 -- "Bus 5 "/LConn2
  Three-Phase Series RLC Load10/LConn3 -- "Bus 14 "/RConn3
  Three-Phase Series RLC Load10/LConn2 -- "Bus 14 "/RConn2
  Three-Phase Series RLC Load10/LConn1 -- "Bus 14 "/RConn1
  Three-Phase Series RLC Load9/LConn3 -- "Bus 13 "/RConn3
  Three-Phase Series RLC Load9/LConn2 -- "Bus 13 "/RConn2
  Three-Phase Series RLC Load9/LConn1 -- "Bus 13 "/RConn1
  Three-Phase Series RLC Load8/LConn3 -- "Bus 12 "/RConn3
  Three-Phase Series RLC Load8/LConn2 -- "Bus 12 "/RConn2
  Three-Phase Series RLC Load8/LConn1 -- "Bus 12 "/RConn1
  Three-Phase Series RLC Load7/LConn3 -- "Bus 11 "/RConn3
  "Bus 11 "/RConn2 -- Three-Phase Series RLC Load7/LConn2
  "Bus 11 "/RConn1 -- Three-Phase Series RLC Load7/LConn1
  Three-Phase Series RLC Load6/LConn3 -- "Bus 10 "/RConn3
  Three-Phase Series RLC Load6/LConn2 -- "Bus 10 "/RConn2
  Three-Phase Series RLC Load6/LConn1 -- "Bus 10 "/RConn1
  "Bus 2 "/LConn3 -- Three-Phase Series RLC Load11/LConn3 -- Three-Phase Transformer (Two Windings)1/RConn3
  Three-Phase Series RLC Branch9/LConn1 -- HIF_B8/LConn1 -- Fault_B8/LConn1 -- "Bus 8 "/LConn1
  Three-Phase Series RLC Branch9/LConn2 -- HIF_B8/LConn2 -- Fault_B8/LConn2 -- "Bus 8 "/LConn2
  Three-Phase Series RLC Branch9/LConn3 -- HIF_B8/LConn3 -- Fault_B8/LConn3 -- "Bus 8 "/LConn3
  Three-Phase Series RLC Load1/LConn1 -- "Bus 4 "/LConn1
  Three-Phase Series RLC Branch11/LConn2 -- "Bus 7 "/LConn2
  Three-Phase Series RLC Branch11/LConn1 -- "Bus 7 "/LConn1
  Three-Phase Transformer (Two Windings)5/RConn2 -- "Bus 1 "/LConn2
  Three-Phase Transformer (Two Windings)5/RConn1 -- "Bus 1 "/LConn1
  Generator1/RConn2 -- Three-Phase Transformer (Two Windings)5/LConn2
  Three-Phase Transformer (Two Windings)5/RConn3 -- "Bus 1 "/LConn3
  Three-Phase Series RLC Load12/LConn2 -- Three-Phase Transformer (Two Windings)2/RConn2 -- "Bus 3 "/LConn2
  Three-Phase Series RLC Load12/LConn1 -- Three-Phase Transformer (Two Windings)2/RConn1 -- "Bus 3 "/LConn1
  Synchronous  Compensator/RConn2 -- Three-Phase Transformer (Two Windings)2/LConn2
  Three-Phase Series RLC Load12/LConn3 -- Three-Phase Transformer (Two Windings)2/RConn3 -- "Bus 3 "/LConn3
  "Bus 6 "/LConn2 -- Three-Phase Transformer (Two Windings)3/RConn2 -- Three-Phase Series RLC Load4/LConn2
  "Bus 6 "/LConn1 -- Three-Phase Transformer (Two Windings)3/RConn1 -- Three-Phase Series RLC Load4/LConn1
  Three-Phase Transformer (Two Windings)3/RConn3 -- "Bus 6 "/LConn3 -- Three-Phase Series RLC Load4/LConn3
  "Synchronous  Compensator "/RConn2 -- Three-Phase Transformer (Two Windings)3/LConn2
  "Bus 4 "/RConn3 -- Fault_B4/LConn3 -- HIF_B4/LConn3 -- Three-Phase Series RLC Branch1/LConn3 -- Three-Phase Series RLC Branch5/RConn3 -- Three-Phase Series RLC Branch6/RConn3 -- Three-Phase Series RLC Branch10/LConn3 -- Three-Phase Series RLC Branch8/RConn3
  "Bus 4 "/RConn2 -- Fault_B4/LConn2 -- HIF_B4/LConn2 -- Three-Phase Series RLC Branch1/LConn2 -- Three-Phase Series RLC Branch6/RConn2 -- Three-Phase Series RLC Branch10/LConn2 -- Three-Phase Series RLC Branch8/RConn2 -- Three-Phase Series RLC Branch5/RConn2
  "Bus 4 "/RConn1 -- HIF_B4/LConn1 -- Three-Phase Series RLC Branch1/LConn1 -- Three-Phase Series RLC Branch6/RConn1 -- Three-Phase Series RLC Branch10/LConn1 -- Three-Phase Series RLC Branch8/RConn1 -- Three-Phase Series RLC Branch5/RConn1 -- Fault_B4/LConn1
  Synchronous Compensator/RConn2 -- Three-Phase Transformer (Two Windings)4/RConn2
  Synchronous Compensator/RConn3 -- Three-Phase Transformer (Two Windings)4/RConn3
  Synchronous Compensator/RConn1 -- Three-Phase Transformer (Two Windings)4/RConn1
  "Synchronous  Compensator "/RConn1 -- Three-Phase Transformer (Two Windings)3/LConn1
  "Synchronous  Compensator "/RConn3 -- Three-Phase Transformer (Two Windings)3/LConn3
  Generator1/RConn3 -- Three-Phase Transformer (Two Windings)5/LConn3
  Generator1/RConn1 -- Three-Phase Transformer (Two Windings)5/LConn1
  Synchronous  Compensator/RConn3 -- Three-Phase Transformer (Two Windings)2/LConn3
  Synchronous  Compensator/RConn1 -- Three-Phase Transformer (Two Windings)2/LConn1
  Generator/RConn1 -- Three-Phase Transformer (Two Windings)1/LConn1
  Generator/RConn3 -- Three-Phase Transformer (Two Windings)1/LConn3
  "Bus 3 "/RConn3 -- HIF_B3/LConn3 -- Fault_B3/LConn3 -- Three-Phase Series RLC Branch5/LConn3 -- Three-Phase Series RLC Branch3/RConn3
  Three-Phase Series RLC Branch19/RConn1 -- M_11/LConn1
  Three-Phase Series RLC Branch19/RConn2 -- M_11/LConn2
  Three-Phase Series RLC Branch19/RConn3 -- M_11/LConn3
  M_11/RConn3 -- "Bus 11 "/LConn3 -- HIF_B11/LConn3 -- Fault_B11/LConn3 -- Three-Phase Series RLC Branch18/RConn3
  M_11/RConn2 -- HIF_B11/LConn2 -- Fault_B11/LConn2 -- "Bus 11 "/LConn2 -- Three-Phase Series RLC Branch18/RConn2
  M_11/RConn1 -- HIF_B11/LConn1 -- Fault_B11/LConn1 -- "Bus 11 "/LConn1 -- Three-Phase Series RLC Branch18/RConn1
  Three-Phase Series RLC Branch16/LConn3 -- M_14/LConn3
  Three-Phase Series RLC Branch16/LConn2 -- M_14/LConn2
  Three-Phase Series RLC Branch16/LConn1 -- M_14/LConn1

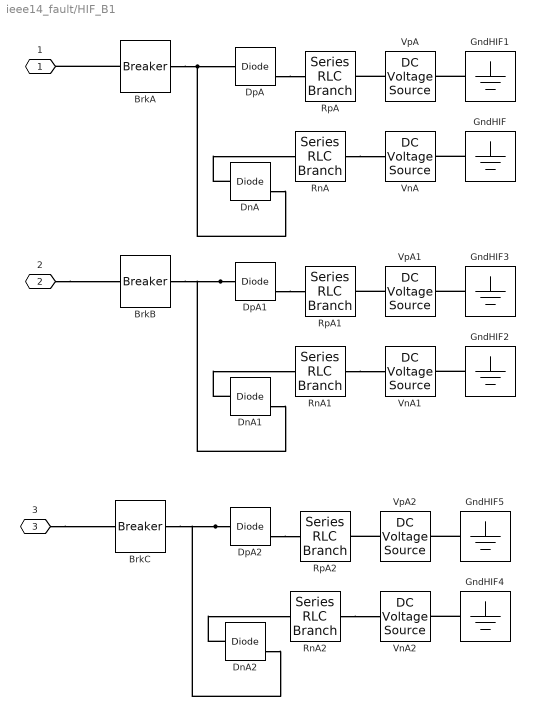
== system ieee14_fault/HIF_B1 ==
  BrkA : spsBreakerLib/Breaker  InitialState=0  SwitchingTimes=[100]  External=off  BreakerResistance=0.01  SnubberResistance=1e6  SnubberCapacitance=inf  Measurements=None  MoreParameters=on  NoBreakLoop=off
  BrkB : spsBreakerLib/Breaker  InitialState=0  SwitchingTimes=[100]  External=off  BreakerResistance=0.01  SnubberResistance=1e6  SnubberCapacitance=inf  Measurements=None  MoreParameters=on  NoBreakLoop=off
  BrkC : spsBreakerLib/Breaker  InitialState=0  SwitchingTimes=[100]  External=off  BreakerResistance=0.01  SnubberResistance=1e6  SnubberCapacitance=inf  Measurements=None  MoreParameters=on  NoBreakLoop=off
  DnA : spsDiodeLib/Diode  Ron=0.001  Lon=0  Vf=0.8  IC=0  UseSnubber=0  Rs=1e6  Cs=inf  Measurements=on
  DnA1 : spsDiodeLib/Diode  Ron=0.001  Lon=0  Vf=0.8  IC=0  UseSnubber=0  Rs=1e6  Cs=inf  Measurements=on
  DnA2 : spsDiodeLib/Diode  Ron=0.001  Lon=0  Vf=0.8  IC=0  UseSnubber=0  Rs=1e6  Cs=inf  Measurements=on
  DpA : spsDiodeLib/Diode  Ron=0.001  Lon=0  Vf=0.8  IC=0  UseSnubber=0  Rs=1e6  Cs=inf  Measurements=on
  DpA1 : spsDiodeLib/Diode  Ron=0.001  Lon=0  Vf=0.8  IC=0  UseSnubber=0  Rs=1e6  Cs=inf  Measurements=on
  DpA2 : spsDiodeLib/Diode  Ron=0.001  Lon=0  Vf=0.8  IC=0  UseSnubber=0  Rs=1e6  Cs=inf  Measurements=on
  GndHIF{,1..5} (6 alike) : spsGroundLib/Ground  LConnTagsString=a
  RnA : spsSeriesRLCBranchLib/Series RLC Branch  LConnTagsString=__new0  RConnTagsString=__new0  BranchType=R  Resistance=160  Inductance=1e-3  SetiL0=off  InitialCurrent=0  Capacitance=1e-6  Setx0=off  InitialVoltage=0  Measurements=None
  RnA1 : spsSeriesRLCBranchLib/Series RLC Branch  LConnTagsString=__new0  RConnTagsString=__new0  BranchType=R  Resistance=160  Inductance=1e-3  SetiL0=off  InitialCurrent=0  Capacitance=1e-6  Setx0=off  InitialVoltage=0  Measurements=None
  RnA2 : spsSeriesRLCBranchLib/Series RLC Branch  LConnTagsString=__new0  RConnTagsString=__new0  BranchType=R  Resistance=160  Inductance=1e-3  SetiL0=off  InitialCurrent=0  Capacitance=1e-6  Setx0=off  InitialVoltage=0  Measurements=None
  RpA : spsSeriesRLCBranchLib/Series RLC Branch  LConnTagsString=__new0  RConnTagsString=__new0  BranchType=R  Resistance=150  Inductance=1e-3  SetiL0=off  InitialCurrent=0  Capacitance=1e-6  Setx0=off  InitialVoltage=0  Measurements=None
  RpA1 : spsSeriesRLCBranchLib/Series RLC Branch  LConnTagsString=__new0  RConnTagsString=__new0  BranchType=R  Resistance=150  Inductance=1e-3  SetiL0=off  InitialCurrent=0  Capacitance=1e-6  Setx0=off  InitialVoltage=0  Measurements=None
  RpA2 : spsSeriesRLCBranchLib/Series RLC Branch  LConnTagsString=__new0  RConnTagsString=__new0  BranchType=R  Resistance=150  Inductance=1e-3  SetiL0=off  InitialCurrent=0  Capacitance=1e-6  Setx0=off  InitialVoltage=0  Measurements=None
  VnA : spsDCVoltageSourceLib/DC Voltage Source  Amplitude=2050  Measurements=None
  VnA1 : spsDCVoltageSourceLib/DC Voltage Source  Amplitude=2050  Measurements=None
  VnA2 : spsDCVoltageSourceLib/DC Voltage Source  Amplitude=2050  Measurements=None
  VpA : spsDCVoltageSourceLib/DC Voltage Source  Amplitude=2000  Measurements=None
  VpA1 : spsDCVoltageSourceLib/DC Voltage Source  Amplitude=2000  Measurements=None
  VpA2 : spsDCVoltageSourceLib/DC Voltage Source  Amplitude=2000  Measurements=None
  1 : PMIOPort  Side=Left
  2 : PMIOPort  Port=2  Side=Left
  3 : PMIOPort  Port=3  Side=Left
  connections:
  GndHIF3/LConn1 -- VpA1/LConn1
  DpA1/LConn1 -- BrkB/RConn1 -- DnA1/RConn1
  GndHIF5/LConn1 -- VpA2/LConn1
  VpA/RConn1 -- RpA/RConn1
  BrkA/LConn1 -- 1/RConn1
  DnA/LConn1 -- RnA/LConn1
  RnA1/RConn1 -- VnA1/LConn1
  DpA2/LConn1 -- BrkC/RConn1 -- DnA2/RConn1
  RnA2/RConn1 -- VnA2/LConn1
  VpA1/RConn1 -- RpA1/RConn1
  GndHIF2/LConn1 -- VnA1/RConn1
  DnA1/LConn1 -- RnA1/LConn1
  DpA2/RConn1 -- RpA2/LConn1
  GndHIF4/LConn1 -- VnA2/RConn1
  RnA/RConn1 -- VnA/LConn1
  VpA2/RConn1 -- RpA2/RConn1
  DnA2/LConn1 -- RnA2/LConn1
  DpA1/RConn1 -- RpA1/LConn1
  BrkA/RConn1 -- DnA/RConn1 -- DpA/LConn1
  GndHIF1/LConn1 -- VpA/LConn1
  DpA/RConn1 -- RpA/LConn1
  GndHIF/LConn1 -- VnA/RConn1
  2/RConn1 -- BrkB/LConn1
  3/RConn1 -- BrkC/LConn1

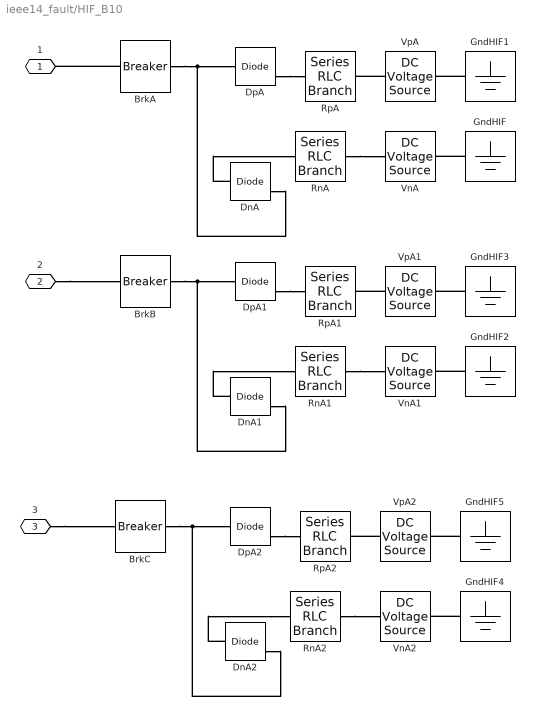
== system ieee14_fault/HIF_B10 ==
  BrkA : spsBreakerLib/Breaker  InitialState=0  SwitchingTimes=[100]  External=off  BreakerResistance=0.01  SnubberResistance=1e6  SnubberCapacitance=inf  Measurements=None  MoreParameters=on  NoBreakLoop=off
  BrkB : spsBreakerLib/Breaker  InitialState=0  SwitchingTimes=[100]  External=off  BreakerResistance=0.01  SnubberResistance=1e6  SnubberCapacitance=inf  Measurements=None  MoreParameters=on  NoBreakLoop=off
  BrkC : spsBreakerLib/Breaker  InitialState=0  SwitchingTimes=[100]  External=off  BreakerResistance=0.01  SnubberResistance=1e6  SnubberCapacitance=inf  Measurements=None  MoreParameters=on  NoBreakLoop=off
  DnA : spsDiodeLib/Diode  Ron=0.001  Lon=0  Vf=0.8  IC=0  UseSnubber=0  Rs=1e6  Cs=inf  Measurements=on
  DnA1 : spsDiodeLib/Diode  Ron=0.001  Lon=0  Vf=0.8  IC=0  UseSnubber=0  Rs=1e6  Cs=inf  Measurements=on
  DnA2 : spsDiodeLib/Diode  Ron=0.001  Lon=0  Vf=0.8  IC=0  UseSnubber=0  Rs=1e6  Cs=inf  Measurements=on
  DpA : spsDiodeLib/Diode  Ron=0.001  Lon=0  Vf=0.8  IC=0  UseSnubber=0  Rs=1e6  Cs=inf  Measurements=on
  DpA1 : spsDiodeLib/Diode  Ron=0.001  Lon=0  Vf=0.8  IC=0  UseSnubber=0  Rs=1e6  Cs=inf  Measurements=on
  DpA2 : spsDiodeLib/Diode  Ron=0.001  Lon=0  Vf=0.8  IC=0  UseSnubber=0  Rs=1e6  Cs=inf  Measurements=on
  GndHIF{,1..5} (6 alike) : spsGroundLib/Ground  LConnTagsString=a
  RnA : spsSeriesRLCBranchLib/Series RLC Branch  LConnTagsString=__new0  RConnTagsString=__new0  BranchType=R  Resistance=160  Inductance=1e-3  SetiL0=off  InitialCurrent=0  Capacitance=1e-6  Setx0=off  InitialVoltage=0  Measurements=None
  RnA1 : spsSeriesRLCBranchLib/Series RLC Branch  LConnTagsString=__new0  RConnTagsString=__new0  BranchType=R  Resistance=160  Inductance=1e-3  SetiL0=off  InitialCurrent=0  Capacitance=1e-6  Setx0=off  InitialVoltage=0  Measurements=None
  RnA2 : spsSeriesRLCBranchLib/Series RLC Branch  LConnTagsString=__new0  RConnTagsString=__new0  BranchType=R  Resistance=160  Inductance=1e-3  SetiL0=off  InitialCurrent=0  Capacitance=1e-6  Setx0=off  InitialVoltage=0  Measurements=None
  RpA : spsSeriesRLCBranchLib/Series RLC Branch  LConnTagsString=__new0  RConnTagsString=__new0  BranchType=R  Resistance=150  Inductance=1e-3  SetiL0=off  InitialCurrent=0  Capacitance=1e-6  Setx0=off  InitialVoltage=0  Measurements=None
  RpA1 : spsSeriesRLCBranchLib/Series RLC Branch  LConnTagsString=__new0  RConnTagsString=__new0  BranchType=R  Resistance=150  Inductance=1e-3  SetiL0=off  InitialCurrent=0  Capacitance=1e-6  Setx0=off  InitialVoltage=0  Measurements=None
  RpA2 : spsSeriesRLCBranchLib/Series RLC Branch  LConnTagsString=__new0  RConnTagsString=__new0  BranchType=R  Resistance=150  Inductance=1e-3  SetiL0=off  InitialCurrent=0  Capacitance=1e-6  Setx0=off  InitialVoltage=0  Measurements=None
  VnA : spsDCVoltageSourceLib/DC Voltage Source  Amplitude=2050  Measurements=None
  VnA1 : spsDCVoltageSourceLib/DC Voltage Source  Amplitude=2050  Measurements=None
  VnA2 : spsDCVoltageSourceLib/DC Voltage Source  Amplitude=2050  Measurements=None
  VpA : spsDCVoltageSourceLib/DC Voltage Source  Amplitude=2000  Measurements=None
  VpA1 : spsDCVoltageSourceLib/DC Voltage Source  Amplitude=2000  Measurements=None
  VpA2 : spsDCVoltageSourceLib/DC Voltage Source  Amplitude=2000  Measurements=None
  1 : PMIOPort  Side=Left
  2 : PMIOPort  Port=2  Side=Left
  3 : PMIOPort  Port=3  Side=Left
  connections:
  GndHIF3/LConn1 -- VpA1/LConn1
  DnA1/RConn1 -- DpA1/LConn1 -- BrkB/RConn1
  GndHIF5/LConn1 -- VpA2/LConn1
  VpA/RConn1 -- RpA/RConn1
  BrkA/LConn1 -- 1/RConn1
  DnA/LConn1 -- RnA/LConn1
  RnA1/RConn1 -- VnA1/LConn1
  DnA2/RConn1 -- DpA2/LConn1 -- BrkC/RConn1
  RnA2/RConn1 -- VnA2/LConn1
  VpA1/RConn1 -- RpA1/RConn1
  GndHIF2/LConn1 -- VnA1/RConn1
  DnA1/LConn1 -- RnA1/LConn1
  DpA2/RConn1 -- RpA2/LConn1
  GndHIF4/LConn1 -- VnA2/RConn1
  RnA/RConn1 -- VnA/LConn1
  VpA2/RConn1 -- RpA2/RConn1
  DnA2/LConn1 -- RnA2/LConn1
  DpA1/RConn1 -- RpA1/LConn1
  BrkA/RConn1 -- DpA/LConn1 -- DnA/RConn1
  GndHIF1/LConn1 -- VpA/LConn1
  DpA/RConn1 -- RpA/LConn1
  GndHIF/LConn1 -- VnA/RConn1
  2/RConn1 -- BrkB/LConn1
  3/RConn1 -- BrkC/LConn1
